simulink model "UAV3_Navigation_01"  (R2026b)
settings: Solver=FixedStepDiscrete  FixedStep=0.1
settings Model: Creator=Ivan  LastModifiedBy=Ivan

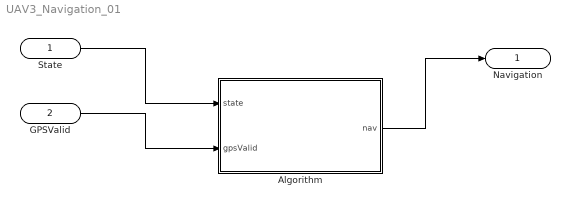
== system UAV3_Navigation_01 ==
  State : Inport  OutDataTypeStr=double  PortDimensions=[5 1]
  GPSValid : Inport  Port=2  OutDataTypeStr=double  PortDimensions=1
  Algorithm : MATLAB Function  TreatAsAtomicUnit=on
  Navigation : Outport
  wires:
  State/1 -> Algorithm/1(state)
  GPSValid/1 -> Algorithm/2(gpsValid)
  Algorithm/1(nav) -> Navigation/1

== matlab function UAV3_Navigation_01/Algorithm ==
  data: state input; nav output; gpsValid input
function nav = v3_navigation(state,gpsValid)
%V3_NAVIGATION Codegen-compatible XY observer with simulated GPS outage.
% state [x;y;vx;vy;battery]; GPS valid = scalar 0/1.
% This is an educational estimator, NOT real GPS/IMU sensor fusion.
%#codegen
persistent lastEstimate
if isempty(lastEstimate)
    lastEstimate = zeros(4,1);
end
if gpsValid >= 0.5 && all(isfinite(state(1:4)))
    nav = 0.9*state(1:4) + 0.1*lastEstimate;
else
    nav = [lastEstimate(1:2)+0.1*lastEstimate(3:4); ...
        lastEstimate(3:4)];
end
lastEstimate = nav;
end
